simulink model "FsaeDynoFull"  (R2026a)
settings: Solver=FixedStepDiscrete  StopTime=t_stop  FixedStep=Ts  EnableMultiTasking=on
PreLoadFcn:
  | FsaeDynoFullData;
InitFcn:
  | FsaeDynoFullData;
values from neighbouring files (symbols this model uses):
  ce = 100    [FsaeDynoFullData.m]
  k_pre = 0.95    [FsaeDynoFullData.m]    (also in FsaeDynoFullPlot.m = evalin('base','k_pre'))
  Ki_id = Rs*wc_dut    (= 13.3454855924)    [FsaeDynoFullData.m]
  Ki_ids = Rs_y*wc_load    (= 47.1238898038)    [FsaeDynoFullData.m]
  Ki_iq = Rs*wc_dut    (= 13.3454855924)    [FsaeDynoFullData.m]
  Ki_iqs = Rs_y*wc_load    (= 47.1238898038)    [FsaeDynoFullData.m]
  Kp_id = Ld*wc_dut    (= 0.102541584213)    [FsaeDynoFullData.m]
  Kp_ids = Ld_y*wc_load    (= 0.204203522483)    [FsaeDynoFullData.m]
  Kp_iq = Lq*wc_dut    (= 0.105557513161)    [FsaeDynoFullData.m]
  Kp_iqs = Lq_y*wc_load    (= 0.204203522483)    [FsaeDynoFullData.m]
  Ld = 40.8e-6    (= 4.08e-05)    [FsaeDynoFullData.m]
  Lq = 42.0e-6    (= 4.2e-05)    [FsaeDynoFullData.m]
  p = 10    [FsaeDynoFullData.m]    (also in buildFsaeDynoFull.m = get_param(ss,'PortHandles'))
  psim = 0.03095    [FsaeDynoFullData.m]
  R_dis_dut = 1/G_dis_dut  - R_disRly    [FsaeDynoFullData.m]
  R_dis_load = 1/G_dis_load - R_disRly    [FsaeDynoFullData.m]
  R_pre_dut = fzero(@(R) preErr(R, Cdc_dut,  G_leak_dut  + G_disRlyOff), [1 1e5])    [FsaeDynoFullData.m]
  R_pre_load = fzero(@(R) preErr(R, Cdc_load, G_leak_load + G_disRlyOff), [1 1e5])    [FsaeDynoFullData.m]
  R_stby_dut = 50e3    (= 50000)    [FsaeDynoFullData.m]
  R_stby_load = 50e3    (= 50000)    [FsaeDynoFullData.m]
  t_InvEnDelay = 0.05    [FsaeDynoFullData.m]
  t_TSoff = t_test + 0.8 + 0.7    (= 2.7)    [FsaeDynoFullData.m]    (also in FsaeDynoFullPlot.m = evalin('base','t_TSoff'))
  Ts = 1e-5    (= 1e-05)    [FsaeDynoFullData.m]
  VbattMin = 50    [FsaeDynoFullData.m]
  VDC_VECT = Vnom*[0.9 1.0 1.1]    [FsaeDynoFullData.m]
  Vnom2 = 400    [FsaeDynoFullData.m]
libraries: nesl_utility x37, fl_lib x22, ee_lib x22, simulink x4, eeTransforms x2, batteryecm_lib x2, eePmsmFieldOrientedControl x1, eePmsmCurrentController x1, eePmsmCurrentReferenceGen x1, eePmsmTorqueEstimator x1, eePwmGeneratorTwoLevel x1
(part 1 of 2)
CloseFcn:
  | clear simlog_FsaeDyno
  | clear logsout_FsaeDyno
Description:
  | Electric Engine Dyno
settings Model: Creator=The MathWorks, Inc.  LastModifiedBy=micha
settings DataIOCC: MaxDataPoints=90000  SignalLoggingName=logsout_FsaeDynoFull
settings SimscapeCC: SimscapeNominalValues="[{\"value\":\"1\",\"unit\":\"A\"},{\"value\":\"1\",\"unit\":\"bar\"},{\"value\":\"1\",\"unit\":\"cm^2\"},{\"value\":\"1\",\"unit\":\"cm^3/s\"},{\"value\":\"1\",\"unit\":\"kJ/kg\"},{\"value\":\"1\",\"unit\":\"kW\"},{\"value\":\"1\",\"unit\":\"l\"},{\"value\":\"1\",\"unit\":\"N\"},{\"value\":\"1\",\"unit\":\"N*m\"},{\"value\":\"1\",\"unit\":\"V\"}]"  SimscapeLogSimulationStatistics=on  SimscapeLogName=simlog_FsaeDyno  SimscapeLogDataHistory=90000.0

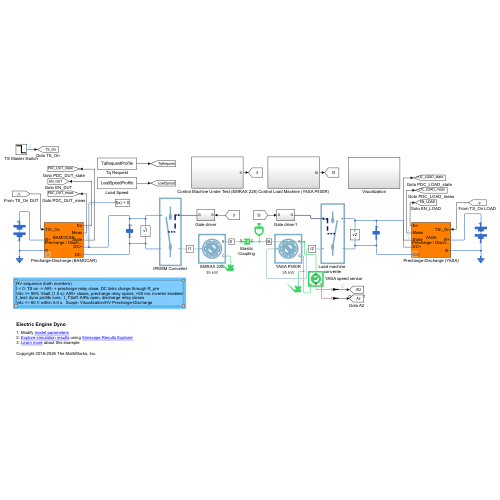
[thumbnail: Simulink's stored preview of the top-level diagram]
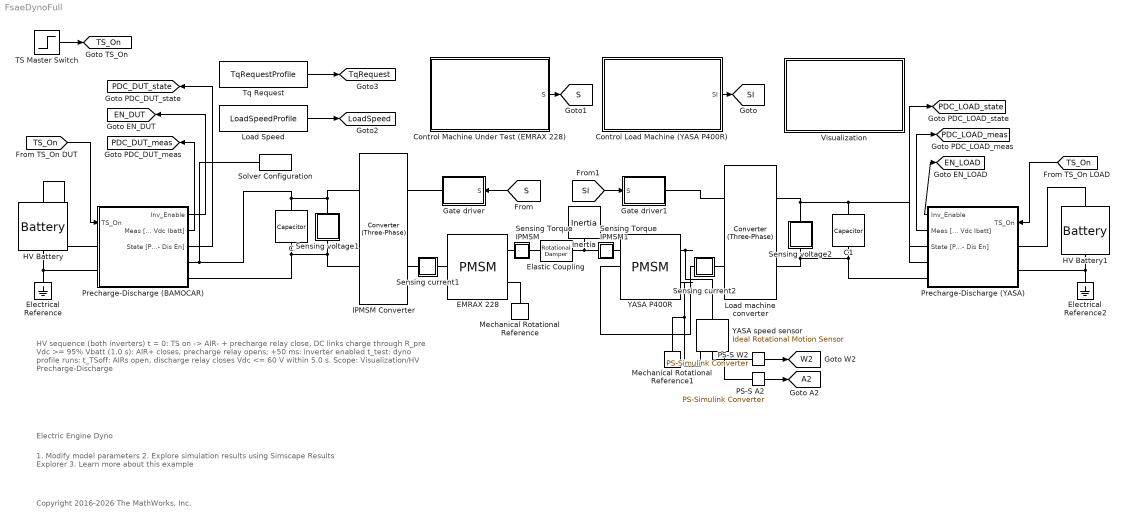
== system FsaeDynoFull ==
  note: Electric Engine Dyno
  note: 1. Modify model parameters
      | 2. Explore simulation results using Simscape Results Explorer
      | 3. Learn more about this example
  note: Copyright 2016-2026 The MathWorks, Inc.
  note: HV sequence (both inverters)
      | t = 0: TS on -> AIR- + precharge relay close, DC links charge through R_pre
      | Vdc >= 95% Vbatt (1.0 s): AIR+ closes, precharge relay opens; +50 ms: inverter enabled
      | t_test: dyno profile runs;  t_TSoff: AIRs open, discharge relay closes
      | Vdc <= 60 V within 5.0 s.  Scope: Visualization/HV Precharge-Discharge
  C : fl_lib/Electrical/Electrical Elements/Capacitor  c=Cdc_dut F  r=1e-6 Ohm  g=0 1/Ohm  i_specify=off  i_priority=None  i=0 A  i_nominal_specify=off  i_nominal_value=1  i_nominal_unit=A  v_specify=off  v_priority=None  v=0 V  v_nominal_specify=off  v_nominal_value=1  v_nominal_unit=V  vc_specify=on  vc_priority=None  vc=0 V  vc_nominal_specify=off  vc_nominal_value=1  vc_nominal_unit=V
  C1 : fl_lib/Electrical/Electrical Elements/Capacitor  c=Cdc_load F  r=1e-6 Ohm  g=0 1/Ohm  i_specify=off  i_priority=None  i=0 A  i_nominal_specify=off  i_nominal_value=1  i_nominal_unit=A  v_specify=off  v_priority=None  v=0 V  v_nominal_specify=off  v_nominal_value=1  v_nominal_unit=V  vc_specify=on  vc_priority=None  vc=0 V  vc_nominal_specify=off  vc_nominal_value=1  vc_nominal_unit=V
  Control Load Machine (YASA P400R) : Subsystem
  Control Machine Under Test (EMRAX 228) : Subsystem
  EMRAX 228 : ee_lib/Electromechanical/Permanent Magnet/PMSM  port_option=ee.enum.threePhasePort.composite  winding_type=ee.enum.statorconnection.wye  machine_param=ee.enum.pmsm.parameterization.constant  nPolePairs=p  pmflux_param=1  pm_flux_linkage=psim Wb  torque_constant=0.18 N*m/A  back_emf_constant=0.18 V/(rad/s)  stator_param=1  Ld=Ld H  Lq=Lq H  idVec=[-200, 0, 200] A  iqVec=[-200, 0, 200] A  LdMatrix=0.0002 * ones(3, 3) H  LqMatrix=0.0002 * ones(3, 3) H  PmMatrix=0.1 * ones(3, 3) Wb  ktMatrix=0.18 * ones(3, 3) N*m/A  keMatrix=0.18 * ones(3, 3) V/(rad/s)  L0=L0 H  Ls=0.0002 H  Lm=0.00002 H  Ms=0.00002 H  Rs=Rs Ohm  zero_sequence=ee.enum.park.zerosequence.exclude  axes_param=ee.enum.rotorangle.qaxis  loss_param=ee.enum.ironloss.none  losses_oc=[0, 0, 0] W  losses_sc=[0, 0, 0] W  f_losses=60 Hz  Isc_losses=95 A  J=0 kg*m^2  lam=0 N*m/(rad/s)  i_d_specify=on  i_d_priority=None  i_d=0 A  i_d_nominal_specify=off  i_d_nominal_value=1  i_d_nominal_unit=A  i_q_specify=on  i_q_priority=None  i_q=0 A  i_q_nominal_specify=off  i_q_nominal_value=1  i_q_nominal_unit=A  torque_specify=off  torque_priority=None  torque=0 N*m  torque_nominal_specify=off  torque_nominal_value=1  torque_nominal_unit=N*m  angular_velocity_specify=off  angular_velocity_priority=None  angular_velocity=0 rpm  angular_velocity_nominal_specify=off  angular_velocity_nominal_value=1  angular_velocity_nominal_unit=rpm  angular_position_specify=on  angular_position_priority=High  angular_position=0 deg  angular_position_nominal_specify=off  angular_position_nominal_value=1  angular_position_nominal_unit=deg  alpha=3.93e-3 1/K  alpha_flux=-0.001 1/K  Tmeas=298.15 K  stator_thermal_mass=100 J/K  rotor_thermal_mass=200 J/K  Rm_percent_rotor=90  Rd_percent_rotor=30  temperatureA_specify=off  temperatureA_priority=High  temperatureA=25 degC  temperatureA_nominal_specify=off  temperatureA_nominal_value=1  temperatureA_nominal_unit=degC  temperatureB_specify=off  temperatureB_priority=High  temperatureB=25 degC  temperatureB_nominal_specify=off  temperatureB_nominal_value=1  temperatureB_nominal_unit=degC  temperatureC_specify=off  temperatureC_priority=High  temperatureC=25 degC  temperatureC_nominal_specify=off  temperatureC_nominal_value=1  temperatureC_nominal_unit=degC  temperatureR_specify=off  temperatureR_priority=High  temperatureR=25 degC  temperatureR_nominal_specify=off  temperatureR_nominal_value=1  temperatureR_nominal_unit=degC
      settings: AttributesFormatString=35 kW
  Elastic Coupling : fl_lib/Mechanical/Rotational Elements/Rotational Damper  D=ce N*m/(rad/s)  w_specify=off  w_priority=None  w=0 rad/s  w_nominal_specify=off  w_nominal_value=1  w_nominal_unit=rad/s  t_specify=off  t_priority=None  t=0 N*m  t_nominal_specify=off  t_nominal_value=1  t_nominal_unit=N*m
      settings: LogSimulationData=on
  Electrical Reference : fl_lib/Electrical/Electrical Elements/Electrical Reference
  Electrical Reference2 : fl_lib/Electrical/Electrical Elements/Electrical Reference
  Gate driver : Subsystem
  Gate driver1 : Subsystem
  HV Battery : batteryecm_lib/Battery  Vnom=Vnom V  prm_dir=1  R1_dis=2 Ohm  R1_ch=2 Ohm  R1=R1_batt Ohm  prm_AH=1  AH=10000 hr*A  V1=V1 V  AH1=3000 hr*A  prm_R2=1  R2=2000 Ohm  Tmeas=298.15 K  charge_measurement_port=simscape.enum.battery.enable.no  prm_dyn=1  Rp1=0.005 Ohm  tau1=30 s  Rp2=0.005 Ohm  tau2=30 s  Rp3=0.005 Ohm  tau3=30 s  Rp4=0.005 Ohm  tau4=30 s  Rp5=0.005 Ohm  tau5=30 s  prm_fade=1  N_fade=100  AH_fade=45 hr*A  R1_fade=2.02 Ohm  R1_ch_fade=2.02 Ohm  V1_fade=10.35 V  prm_age=1  prm_age_OCV=1  OCV_age=0.9  SOC_age=60  Tmeas_age=298.15 K  delta_time_age_vec=[0] d  temperature_age_vec=[273] K  OCV_scaling_age=2.2134e6  OCV_offset_age=1.632e6  temp_exp_age=0.515833569 V  t_exp_age=0.75  Vnom_T2=12 V  R1_T2=2.2 Ohm  R1_T2_dis=2.2 Ohm  R1_T2_ch=2.2 Ohm  V1_T2=11.4 V  R2_T2=2200 Ohm  Rp1_T2=0.005 Ohm  tau1_T2=30 s  Rp2_T2=0.005 Ohm  tau2_T2=30 s  Rp3_T2=0.005 Ohm  tau3_T2=30 s  Rp4_T2=0.005 Ohm  tau4_T2=30 s  Rp5_T2=0.005 Ohm  tau5_T2=30 s  Tmeas2=273.15 K  thermal_port=simscape.enum.thermaleffects.omit  thermal_mass=30000 J/K  i_specify=off  i_priority=None  i=0 A  i_nominal_specify=off  i_nominal_value=1  i_nominal_unit=A  v_specify=off  v_priority=None  v=0 V  v_nominal_specify=off  v_nominal_value=1  v_nominal_unit=V  charge_specify=on  charge_priority=None  charge=8000 hr*A  charge_nominal_specify=off  charge_nominal_value=1  charge_nominal_unit=A*hr  num_cycles_specify=off  num_cycles_priority=High  num_cycles=0  num_cycles_nominal_specify=off  num_cycles_nominal_value=1  num_cycles_nominal_unit=1  temperature_specify=off  temperature_priority=High  temperature=298.15 K  temperature_nominal_specify=off  temperature_nominal_value=1  temperature_nominal_unit=K
  HV Battery1 : batteryecm_lib/Battery  Vnom=Vnom2 V  prm_dir=1  R1_dis=2 Ohm  R1_ch=2 Ohm  R1=R1_batt Ohm  prm_AH=1  AH=25000 hr*A  V1=V1_2 V  AH1=20000 hr*A  prm_R2=1  R2=2000 Ohm  Tmeas=298.15 K  charge_measurement_port=simscape.enum.battery.enable.no  prm_dyn=1  Rp1=0.005 Ohm  tau1=30 s  Rp2=0.005 Ohm  tau2=30 s  Rp3=0.005 Ohm  tau3=30 s  Rp4=0.005 Ohm  tau4=30 s  Rp5=0.005 Ohm  tau5=30 s  prm_fade=1  N_fade=100  AH_fade=45 hr*A  R1_fade=2.02 Ohm  R1_ch_fade=2.02 Ohm  V1_fade=10.35 V  prm_age=1  prm_age_OCV=1  OCV_age=0.9  SOC_age=60  Tmeas_age=298.15 K  delta_time_age_vec=[0] d  temperature_age_vec=[273] K  OCV_scaling_age=2.2134e6  OCV_offset_age=1.632e6  temp_exp_age=0.515833569 V  t_exp_age=0.75  Vnom_T2=12 V  R1_T2=2.2 Ohm  R1_T2_dis=2.2 Ohm  R1_T2_ch=2.2 Ohm  V1_T2=11.4 V  R2_T2=2200 Ohm  Rp1_T2=0.005 Ohm  tau1_T2=30 s  Rp2_T2=0.005 Ohm  tau2_T2=30 s  Rp3_T2=0.005 Ohm  tau3_T2=30 s  Rp4_T2=0.005 Ohm  tau4_T2=30 s  Rp5_T2=0.005 Ohm  tau5_T2=30 s  Tmeas2=273.15 K  thermal_port=simscape.enum.thermaleffects.omit  thermal_mass=30000 J/K  i_specify=off  i_priority=None  i=0 A  i_nominal_specify=off  i_nominal_value=1  i_nominal_unit=A  v_specify=off  v_priority=None  v=0 V  v_nominal_specify=off  v_nominal_value=1  v_nominal_unit=V  charge_specify=on  charge_priority=None  charge=20000 hr*A  charge_nominal_specify=off  charge_nominal_value=1  charge_nominal_unit=A*hr  num_cycles_specify=off  num_cycles_priority=High  num_cycles=0  num_cycles_nominal_specify=off  num_cycles_nominal_value=1  num_cycles_nominal_unit=1  temperature_specify=off  temperature_priority=High  temperature=298.15 K  temperature_nominal_specify=off  temperature_nominal_value=1  temperature_nominal_unit=K
  IPMSM Converter : ee_lib/Semiconductors & Converters/Converters/Converter (Three-Phase)  port_option=ee.enum.threePhasePort.composite  fidelity_option=ee.enum.converters.fidelity.detailed  device_type=3  showThermalPort=false  K=0  Vth=0.5 V  Vgt=1 V  Vgt_off=-1 V  Ih=1 A  Vf=0.8 V  Ron=0.001 Ohm  Rds=0.001 Ohm  Goff=1e-5 1/Ohm  Eon_scalar=22.86e-3 J  Eoff_scalar=17.14e-3 J  Eoff_natural_commutation=10e-3 J  Voff=300 V  Iout_scalar=600 A  onCurrentMeasDelay=0 s  useCurrentFromPreviousCycle=false  useVoltageFromPreviousCycle=false  diode_param=2  diode_Vf=0.8 V  diode_Ron=0.001 Ohm  diode_Goff=1e-5 1/Ohm  diode_C=50 nF  diode_iRM=-235 A  diode_iF=300 A  diode_idot=-50 A/us  diode_trr_param=1  diode_trr_factor=3  diode_trr=15 us  diode_Qrr=1.5e+3 s*uA  diode_rec_loss_model=ee.enum.diode.reverseRecoveryModel.fixed  diode_ErecVal=0 J  diode_scaleWithIandV=false  diode_ErecMat=zeros(2, 3) J  diode_TjrecVec=[298.15, 398.15] K  diode_IfrecVec=[.1, 1, 10] A  diode_IrecVal=10 A  diode_VrecVal=10 V  diode_tFilter=1 / 1000 / 100 s  thermal_network_parameterization=ee.enum.thermalNetworkTopology.external  Rth=[.08, .5] K/W  Rth_Cauer=[.08, .1, .5] K/W  Rth_Foster=[.08, .14, .22, .16] K/W  thermal_mass_parameterization=ee.enum.thermalNetwork.timeconstant  thermal_mass=[.01, .5] J/K  thermal_mass_Cauer=[.01, .1, .5] J/K  thermal_mass_Foster=[.001, .005, .05, .5] J/K  thermal_time_constant=[.001, .2] s  thermal_time_constant_Cauer=[.001, .1, .2] s  thermal_time_constant_Foster=[7e-05, .0007, .01, .08] s  thermal_mass_initial_temperatures=[25, 25] degC  thermal_mass_initial_temperatures_Cauer=[25, 25, 25] degC  junction_thermal_mass=0.01 J/K  Tvec_initial_Foster=[25, 25, 25, 25] degC  snubber_type=0  Cs=1e-7 F  Rs=0.1 Ohm  Vce_loss=[0, 150, 300] V
  Inertia : fl_lib/Mechanical/Rotational Elements/Inertia  inertia=Jm kg*m^2  num_ports=foundation.enum.numPorts2.one  w_specify=off  w_priority=High  w=0 rad/s  w_nominal_specify=off  w_nominal_value=1  w_nominal_unit=rad/s  t_specify=off  t_priority=None  t=0 N*m  t_nominal_specify=off  t_nominal_value=1  t_nominal_unit=N*m
  Load Speed : FromWorkspace  VariableName=LoadSpeedProfile  OutputAfterFinalValue=Holding final value
  Load machine converter : ee_lib/Semiconductors & Converters/Converters/Converter (Three-Phase)  port_option=ee.enum.threePhasePort.composite  fidelity_option=ee.enum.converters.fidelity.detailed  device_type=3  showThermalPort=false  K=0  Vth=0.5 V  Vgt=1 V  Vgt_off=-1 V  Ih=1 A  Vf=0.8 V  Ron=0.001 Ohm  Rds=0.001 Ohm  Goff=1e-5 1/Ohm  Eon_scalar=22.86e-3 J  Eoff_scalar=17.14e-3 J  Eoff_natural_commutation=10e-3 J  Voff=300 V  Iout_scalar=600 A  onCurrentMeasDelay=0 s  useCurrentFromPreviousCycle=false  useVoltageFromPreviousCycle=false  diode_param=2  diode_Vf=0.8 V  diode_Ron=0.001 Ohm  diode_Goff=1e-5 1/Ohm  diode_C=50 nF  diode_iRM=-235 A  diode_iF=300 A  diode_idot=-50 A/us  diode_trr_param=1  diode_trr_factor=3  diode_trr=15 us  diode_Qrr=1.5e+3 s*uA  diode_rec_loss_model=ee.enum.diode.reverseRecoveryModel.fixed  diode_ErecVal=0 J  diode_scaleWithIandV=false  diode_ErecMat=zeros(2, 3) J  diode_TjrecVec=[298.15, 398.15] K  diode_IfrecVec=[.1, 1, 10] A  diode_IrecVal=10 A  diode_VrecVal=10 V  diode_tFilter=1 / 1000 / 100 s  thermal_network_parameterization=ee.enum.thermalNetworkTopology.external  Rth=[.08, .5] K/W  Rth_Cauer=[.08, .1, .5] K/W  Rth_Foster=[.08, .14, .22, .16] K/W  thermal_mass_parameterization=ee.enum.thermalNetwork.timeconstant  thermal_mass=[.01, .5] J/K  thermal_mass_Cauer=[.01, .1, .5] J/K  thermal_mass_Foster=[.001, .005, .05, .5] J/K  thermal_time_constant=[.001, .2] s  thermal_time_constant_Cauer=[.001, .1, .2] s  thermal_time_constant_Foster=[7e-05, .0007, .01, .08] s  thermal_mass_initial_temperatures=[25, 25] degC  thermal_mass_initial_temperatures_Cauer=[25, 25, 25] degC  junction_thermal_mass=0.01 J/K  Tvec_initial_Foster=[25, 25, 25, 25] degC  snubber_type=0  Cs=1e-7 F  Rs=0.1 Ohm  Vce_loss=[0, 150, 300] V
  Mechanical Rotational Reference : fl_lib/Mechanical/Rotational Elements/Mechanical Rotational Reference
  Mechanical Rotational Reference1 : fl_lib/Mechanical/Rotational Elements/Mechanical Rotational Reference
  PS-S A2 : nesl_utility/PS-Simulink Converter  PhysicalDomain=network_engine_domain  SubClassName=ps_output  LeftPortType=input  RightPortType=output  PseudoPeriodic=off  Frequencies=[]  VectorFormat=1-D array  Unit=rad  AffineConversion=off
  PS-S W2 : nesl_utility/PS-Simulink Converter  PhysicalDomain=network_engine_domain  SubClassName=ps_output  LeftPortType=input  RightPortType=output  PseudoPeriodic=off  Frequencies=[]  VectorFormat=1-D array  Unit=rad/s  AffineConversion=off
  Precharge-Discharge (BAMOCAR) : Subsystem  mask(Precharge / Discharge Circuit){Rpre=R_pre_dut, Rdis=R_dis_dut, Rstby=R_stby_dut, kpre=k_pre, tEnable=t_InvEnDelay, VbattMin=VbattMin}
      mask prompts: Rpre "Precharge resistance [Ohm]"; Rdis "Discharge resistance [Ohm]"; Rstby "Standby (bleeder) resistance [Ohm]"; kpre "Precharge-complete threshold [-]"; tEnable "Inverter enable delay after AIR+ [s]"; VbattMin "Minimum valid accumulator voltage [V]"
      mask help:
      | Accumulator isolation (AIR+, AIR-), precharge relay + resistor, inverter-side discharge relay + resistor and bleeder, with the sequencing logic from PrechargeDischargeCircuit_BAMOCAR.
      | TS_On = 1: precharge, close AIR+ at Vdc >= kpre*Vbatt, enable inverter after tEnable.  TS_On = 0: open AIRs, close discharge relay.
      mask Display:
      | disp('BAMOCAR\nPrecharge / Discharge');
      | port_label('LConn',1,'B+'); port_label('LConn',2,'B-');
      | port_label('RConn',1,'DC+'); port_label('RConn',2,'DC-');
      | port_label('input',1,'TS\_On'); port_label('output',1,'En');
      | port_label('output',2,'Meas'); port_label('output',3,'State');
  Precharge-Discharge (YASA) : Subsystem  mask(Precharge / Discharge Circuit){Rpre=R_pre_load, Rdis=R_dis_load, Rstby=R_stby_load, kpre=k_pre, tEnable=t_InvEnDelay, VbattMin=VbattMin}
      mask prompts: Rpre "Precharge resistance [Ohm]"; Rdis "Discharge resistance [Ohm]"; Rstby "Standby (bleeder) resistance [Ohm]"; kpre "Precharge-complete threshold [-]"; tEnable "Inverter enable delay after AIR+ [s]"; VbattMin "Minimum valid accumulator voltage [V]"
      mask help:
      | Accumulator isolation (AIR+, AIR-), precharge relay + resistor, inverter-side discharge relay + resistor and bleeder, with the sequencing logic from PrechargeDischargeCircuit_YASA.
      | TS_On = 1: precharge, close AIR+ at Vdc >= kpre*Vbatt, enable inverter after tEnable.  TS_On = 0: open AIRs, close discharge relay.
      mask Display:
      | disp('YASA\nPrecharge / Discharge');
      | port_label('LConn',1,'B+'); port_label('LConn',2,'B-');
      | port_label('RConn',1,'DC+'); port_label('RConn',2,'DC-');
      | port_label('input',1,'TS\_On'); port_label('output',1,'En');
      | port_label('output',2,'Meas'); port_label('output',3,'State');
  Sensing Torque IPMSM : Subsystem
      mask Display: disp('tI')
  Sensing Torque IPMSM1 : Subsystem
      mask Display: disp('tA')
  Sensing current1 : Subsystem
      mask Display: disp('i1')
  Sensing current2 : Subsystem
      mask Display: disp('i2')
  Sensing voltage1 : Subsystem
      mask Display: disp('v1')
  Sensing voltage2 : Subsystem
      mask Display: disp('v2')
  Solver Configuration : nesl_utility/Solver Configuration  PhysicalDomain=network_engine_domain  SubClassName=solver  LeftPortType=input  RightPortType=generic  Tones=[]  Harmonics=[]  SimulateNoise=off  Profile=off  UseLocalSampling=off  EnableSwitchedLinearOptims=on  FrequencyDomain=off  UseCCode=off  RelTol=0.001  AbsTol=1e-06  MinStep=1e-09  ToWorkspace=off  RevertToSquareIcSolve=off  NumHomotopyIterations=100  PhasorMode=off  PhasorModeNumHarmonics=1  ConsistencySolver=NEWTON_FTOL  CanonicalOrdering=UNORDERED  OptimizeIntermediates=UNOPTIMIZED  IndexReductionMethod=DerivativeReplacement  DoDC=off  ResidualTolerance=1e-9  ConsistencyTolSource=GLOBAL  ConsistencyAbsTol=0.001  ConsistencyRelTol=0.001  ConsistencyTolFactor=0.001  UseLocalSolver=on  LocalSolverChoice=NE_BACKWARD_EULER_ADVANCER  ResolveIndetEquations=on  FunctionEvalNumThread=1  LocalSolverSampleTime=Ts  DoFixedCost=on  MaxNonlinIter=5  MaxModeIter=2  ComputeImpulses=off  ImpulseIterations=2  LinearAlgebra=auto  LinearAlgebraNumThread=0  EquationFormulation=NE_TIME_EF  DelaysMemoryBudget=1024  AutomaticFiltering=on  FilteringTimeConstant=0.001  PartitionStorageMethod=AS_NEEDED  PartitionMemoryBudget=1024  PartitionMethod=FAST  MultibodyUseLocalSolver=off  MultibodyLocalSolverChoice=ODE1  MultibodyLocalSolverSampleTime=0.001
  TS Master Switch : Step  Time=t_TSoff  InitialValue=1  FinalValue=0  SampleTime=Ts
  Tq Request : FromWorkspace  VariableName=TqRequestProfile  OutputAfterFinalValue=Holding final value
  Visualization : Subsystem
  YASA P400R : ee_lib/Electromechanical/Permanent Magnet/PMSM  port_option=ee.enum.threePhasePort.composite  winding_type=ee.enum.statorconnection.wye  machine_param=ee.enum.pmsm.parameterization.constant  nPolePairs=p_y  pmflux_param=1  pm_flux_linkage=psim_y Wb  torque_constant=0.18 N*m/A  back_emf_constant=0.18 V/(rad/s)  stator_param=1  Ld=Ld_y H  Lq=Lq_y H  idVec=[-200, 0, 200] A  iqVec=[-200, 0, 200] A  LdMatrix=0.0002 * ones(3, 3) H  LqMatrix=0.0002 * ones(3, 3) H  PmMatrix=0.1 * ones(3, 3) Wb  ktMatrix=0.18 * ones(3, 3) N*m/A  keMatrix=0.18 * ones(3, 3) V/(rad/s)  L0=Ld_y H  Ls=0.0002 H  Lm=0.00002 H  Ms=0.00002 H  Rs=Rs_y Ohm  zero_sequence=ee.enum.park.zerosequence.exclude  axes_param=ee.enum.rotorangle.qaxis  loss_param=ee.enum.ironloss.none  losses_oc=[0, 0, 0] W  losses_sc=[0, 0, 0] W  f_losses=60 Hz  Isc_losses=95 A  J=0 kg*m^2  lam=0 N*m/(rad/s)  i_d_specify=on  i_d_priority=None  i_d=0 A  i_d_nominal_specify=off  i_d_nominal_value=1  i_d_nominal_unit=A  i_q_specify=on  i_q_priority=None  i_q=0 A  i_q_nominal_specify=off  i_q_nominal_value=1  i_q_nominal_unit=A  torque_specify=off  torque_priority=None  torque=0 N*m  torque_nominal_specify=off  torque_nominal_value=1  torque_nominal_unit=N*m  angular_velocity_specify=off  angular_velocity_priority=None  angular_velocity=0 rpm  angular_velocity_nominal_specify=off  angular_velocity_nominal_value=1  angular_velocity_nominal_unit=rpm  angular_position_specify=on  angular_position_priority=High  angular_position=0 deg  angular_position_nominal_specify=off  angular_position_nominal_value=1  angular_position_nominal_unit=deg  alpha=3.93e-3 1/K  alpha_flux=-0.001 1/K  Tmeas=298.15 K  stator_thermal_mass=100 J/K  rotor_thermal_mass=200 J/K  Rm_percent_rotor=90  Rd_percent_rotor=30  temperatureA_specify=off  temperatureA_priority=High  temperatureA=25 degC  temperatureA_nominal_specify=off  temperatureA_nominal_value=1  temperatureA_nominal_unit=degC  temperatureB_specify=off  temperatureB_priority=High  temperatureB=25 degC  temperatureB_nominal_specify=off  temperatureB_nominal_value=1  temperatureB_nominal_unit=degC  temperatureC_specify=off  temperatureC_priority=High  temperatureC=25 degC  temperatureC_nominal_specify=off  temperatureC_nominal_value=1  temperatureC_nominal_unit=degC  temperatureR_specify=off  temperatureR_priority=High  temperatureR=25 degC  temperatureR_nominal_specify=off  temperatureR_nominal_value=1  temperatureR_nominal_unit=degC
      settings: AttributesFormatString=35 kW
  YASA speed sensor : fl_lib/Mechanical/Mechanical Sensors/Ideal Rotational Motion Sensor  reference=foundation.enum.MeasurementReference.difference  acceleration_port=false  velocity_port=true  position_port=true  wrap_angle=simscape.enum.onoff.off  offset=0 deg
  tag scope: A2=global, EN_DUT=global, EN_LOAD=global, LoadSpeed=global, PDC_DUT_meas=global, PDC_DUT_state=global, PDC_LOAD_meas=global, PDC_LOAD_state=global, S=global, SI=global, TS_On=global, TqRequest=global, W2=global
  wires:
  [S] -> Gate driver/1(S)
  Control Load Machine (YASA P400R)/1(SI) -> [SI]
  Control Machine Under Test (EMRAX 228)/1(S) -> [S]
  [SI] -> Gate driver1/1(S)
  PS-S W2/1 -> [W2]
  PS-S A2/1 -> [A2]
  Load Speed/1 -> [LoadSpeed]
  Tq Request/1 -> [TqRequest]
  TS Master Switch/1 -> [TS_On]
  [TS_On] -> Precharge-Discharge (BAMOCAR)/1(TS_On)
  Precharge-Discharge (BAMOCAR)/1(Inv_Enable) -> [EN_DUT]
  Precharge-Discharge (BAMOCAR)/2(Meas [Vbatt Vdc Ibatt]) -> [PDC_DUT_meas]
  Precharge-Discharge (BAMOCAR)/3(State [Pre AIR+ AIR- Dis En]) -> [PDC_DUT_state]
  [TS_On] -> Precharge-Discharge (YASA)/1(TS_On)
  Precharge-Discharge (YASA)/1(Inv_Enable) -> [EN_LOAD]
  Precharge-Discharge (YASA)/2(Meas [Vbatt Vdc Ibatt]) -> [PDC_LOAD_meas]
  Precharge-Discharge (YASA)/3(State [Pre AIR+ AIR- Dis En]) -> [PDC_LOAD_state]
  connections:
  Gate driver/RConn1 -- IPMSM Converter/LConn1
  EMRAX 228/RConn2 -- Mechanical Rotational Reference/LConn1
  Elastic Coupling/LConn1 -- Sensing Torque IPMSM/RConn1
  IPMSM Converter/LConn2 -- Sensing current1/LConn1
  EMRAX 228/LConn1 -- Sensing current1/RConn1
  Sensing current2/LConn1 -- Load machine converter/LConn2
  Gate driver1/RConn1 -- Load machine converter/LConn1
  Elastic Coupling/RConn1 -- Sensing Torque IPMSM1/LConn1 -- Inertia/LConn1
  Sensing Torque IPMSM/LConn1 -- EMRAX 228/RConn1
  YASA P400R/LConn1 -- Sensing current2/RConn1
  Sensing Torque IPMSM1/RConn1 -- YASA P400R/RConn1 -- YASA speed sensor/LConn1
  Mechanical Rotational Reference1/LConn1 -- YASA P400R/RConn2 -- YASA speed sensor/RConn1
  YASA speed sensor/RConn2 -- PS-S W2/LConn1
  YASA speed sensor/RConn3 -- PS-S A2/LConn1
  HV Battery/LConn1 -- Precharge-Discharge (BAMOCAR)/LConn1
  Precharge-Discharge (BAMOCAR)/LConn2 -- HV Battery/RConn1 -- Electrical Reference/LConn1
  C/LConn1 -- Precharge-Discharge (BAMOCAR)/RConn1 -- Solver Configuration/RConn1 -- Sensing voltage1/LConn1 -- IPMSM Converter/RConn1
  C/RConn1 -- Precharge-Discharge (BAMOCAR)/RConn2 -- Sensing voltage1/RConn1 -- IPMSM Converter/RConn2
  HV Battery1/LConn1 -- Precharge-Discharge (YASA)/LConn1
  Precharge-Discharge (YASA)/LConn2 -- HV Battery1/RConn1 -- Electrical Reference2/LConn1
  C1/LConn1 -- Precharge-Discharge (YASA)/RConn1 -- Sensing voltage2/LConn1 -- Load machine converter/RConn1
  C1/RConn1 -- Precharge-Discharge (YASA)/RConn2 -- Sensing voltage2/RConn1 -- Load machine converter/RConn2

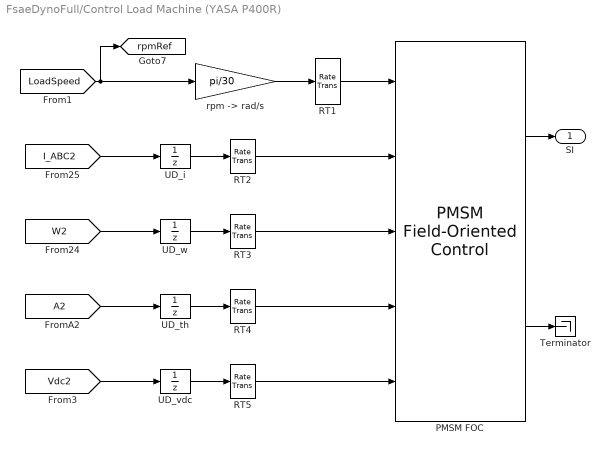
== system FsaeDynoFull/Control Load Machine (YASA P400R) ==
  PMSM FOC : eePmsmFieldOrientedControl/PMSM Field-Oriented Control  winding_type=Wye-wound  CtrlMode=Velocity control  Vnom=Vnom2  Pmax=Pmax_y  Tmax=Tmax_y  p=p_y  Vdc_on=0.5*Vnom2  Ts=Ts  Tsc=Tsc  CtrlType=PI control  Kp_w=Kp_wr  Ki_w=Ki_wr  Kv_w=1  Kaw_w=Kaw_wr  RefType=Zero d-axis control  rpmVec=[0, 3000]  TqVec=[-100, 0, 100]  VdcVec=[300, 350]  PWMMode=SVM: space vector modulation  ModFactor=1  idMatrix=zeros(2,3,2)  iqMatrix=zeros(2,3,2)  psim=psim_y  Ld=Ld_y  Lq=Lq_y  Rs=Rs_y  AxisAlignment=Q-axis  Kp_id=Kp_ids  Ki_id=Ki_ids  Kaw_id=Ki_ids/Kp_ids  Kp_iq=Kp_iqs  Ki_iq=Ki_iqs  Kaw_iq=Ki_iqs/Kp_iqs  AxisPrio=Q-axis  ActZC=off  ActFF=on  ParamTypeFF=Constant parameters  LdFF=Ld_y  LqFF=Lq_y  psimFF=psim_y  idVect=[-200, 0, 200]  iqVect=[-200, 0, 200]  LdMatrix=0.0002 * ones(3, 3)  LqMatrix=0.0002 * ones(3, 3)  psimMatrix=0.04 * ones(3, 3)  CPWMMode=SVM: space vector modulation  fsw=fsw2
  RT{1..5} (5 alike) : RateTransition  OutPortSampleTime=Tsc
  Terminator : Terminator
  UD_i : UnitDelay  SampleTime=Ts
  UD_th : UnitDelay  SampleTime=Ts
  UD_vdc : UnitDelay  SampleTime=Ts
  UD_w : UnitDelay  SampleTime=Ts
  "rpm -> rad/s" : Gain  Gain=pi/30
  SI : Outport  VectorParamsAs1DForOutWhenUnconnected=off
  tag scope: rpmRef=global
  wires:
  [I_ABC2] -> UD_i/1
  [W2] -> UD_w/1
  [A2] -> UD_th/1
  [Vdc2] -> UD_vdc/1
  [LoadSpeed] -> "rpm -> rad/s"/1, [rpmRef]
  PMSM FOC/1 -> SI/1
  PMSM FOC/2 -> Terminator/1
  "rpm -> rad/s"/1 -> RT1/1
  RT1/1 -> PMSM FOC/1
  UD_i/1 -> RT2/1
  RT2/1 -> PMSM FOC/2
  UD_w/1 -> RT3/1
  RT3/1 -> PMSM FOC/3
  UD_th/1 -> RT4/1
  RT4/1 -> PMSM FOC/4
  UD_vdc/1 -> RT5/1
  RT5/1 -> PMSM FOC/5

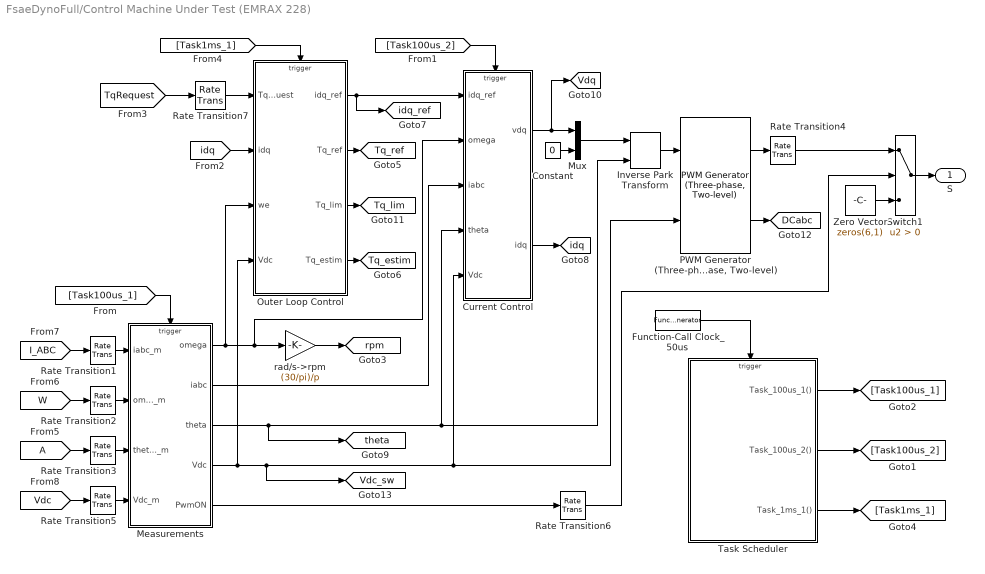
== system FsaeDynoFull/Control Machine Under Test (EMRAX 228) ==
  Constant : Constant  Value=0  SampleTime=-1
  Current Control : Subsystem
  From5 : From  TagVisibility=global
  Function-Call Clock_50us : FunctionCallGenerator  SampleTime=5e-5
  Inverse Park Transform : eeTransforms/Inverse Park Transform  AxisAlignment=Q-axis  PowerInvariant=off
  Measurements : Subsystem
  Mux : Mux  Inputs=2
  Outer Loop Control : Subsystem
  "PWM Generator (Three-phase, Two-level)" : eePwmGeneratorTwoLevel/PWM Generator (Three-phase, Two-level)  PWMMode=Continuous PWM (CPWM)  CPWMMode=SVM: space vector modulation  DPWMMode=60 DPWM: 60 degree discontinuous PWM  fsw=fsw  Ts=Ts
  Rate Transition{1..7} (7 alike) : RateTransition
  Switch1 : Switch  Criteria=u2 > Threshold  SaturateOnIntegerOverflow=off  InputSameDT=off
  Task Scheduler : Stateflow chart  TreatAsAtomicUnit=on
  Zero Vector : Constant  Value=zeros(6,1)  SampleTime=-1
  rad/s->rpm : Gain  Gain=(30/pi)/p
  S : Outport  VectorParamsAs1DForOutWhenUnconnected=off
  tag scope: DCabc=global, Tq_estim=global, Tq_lim=global, Tq_ref=global, Vdc_sw=global, Vdq=global, idq=global, idq_ref=global, rpm=global, theta=global
  wires:
  Current Control/1(vdq) -> [Vdq], Mux/1
  Measurements/2(iabc) -> Current Control/3(iabc)
  Measurements/3(theta) -> [theta], Inverse Park Transform/2, Current Control/4(theta)
  "PWM Generator (Three-phase, Two-level)"/1 -> Rate Transition4/1
  Inverse Park Transform/1 -> "PWM Generator (Three-phase, Two-level)"/1
  [I_ABC] -> Rate Transition1/1
  [W] -> Rate Transition2/1
  From5/1 -> Rate Transition3/1
  [Vdc] -> Rate Transition5/1
  Outer Loop Control/1(idq_ref) -> [idq_ref], Current Control/1(idq_ref)
  "PWM Generator (Three-phase, Two-level)"/2 -> [DCabc]
  Rate Transition1/1 -> Measurements/1(iabc_m)
  Rate Transition2/1 -> Measurements/2(omega_m)
  Rate Transition3/1 -> Measurements/3(theta_m)
  Rate Transition5/1 -> Measurements/4(Vdc_m)
  Function-Call Clock_50us/1 -> Task Scheduler/Trigger
  Task Scheduler/3(Task_1ms_1()) -> [Task1ms_1]
  Task Scheduler/2(Task_100us_2()) -> [Task100us_2]
  Task Scheduler/1(Task_100us_1()) -> [Task100us_1]
  Outer Loop Control/2(Tq_ref) -> [Tq_ref]
  Measurements/1(omega) -> Outer Loop Control/3(we), Current Control/2(omega), rad/s->rpm/1
  rad/s->rpm/1 -> [rpm]
  Outer Loop Control/3(Tq_lim) -> [Tq_lim]
  Rate Transition7/1 -> Outer Loop Control/1(TqRequest)
  [TqRequest] -> Rate Transition7/1
  Outer Loop Control/4(Tq_estim) -> [Tq_estim]
  [idq] -> Outer Loop Control/2(idq)
  Measurements/4(Vdc) -> [Vdc_sw], "PWM Generator (Three-phase, Two-level)"/2, Current Control/5(Vdc), Outer Loop Control/4(Vdc)
  Rate Transition4/1 -> Switch1/1
  Switch1/1 -> S/1
  Measurements/5(PwmON) -> Rate Transition6/1
  Zero Vector/1 -> Switch1/3
  Rate Transition6/1 -> Switch1/2
  [Task100us_2] -> Current Control/Trigger
  [Task1ms_1] -> Outer Loop Control/Trigger
  [Task100us_1] -> Measurements/Trigger
  Current Control/2(idq) -> [idq]
  Constant/1 -> Mux/2
  Mux/1 -> Inverse Park Transform/1

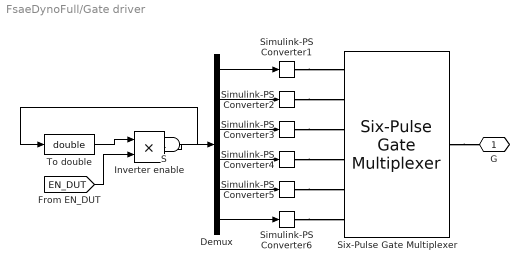
== system FsaeDynoFull/Gate driver ==
  S : Inport
  Demux : Demux  Outputs=6
  Inverter enable : Product  Inputs=**
  Simulink-PS Converter{1..6} (6 alike) : nesl_utility/Simulink-PS Converter  PhysicalDomain=network_engine_domain  SubClassName=ps_input  LeftPortType=input  RightPortType=output  PseudoPeriodic=off  Frequencies=[]  NoiseDistribution=none  NoiseParameters=[]  Unit=1  AffineConversion=off  FilteringAndDerivatives=zero  SimscapeFilterOrder=1  InputFilterTimeConstant=0.001  UdotUserProvided=1
  Six-Pulse Gate Multiplexer : ee_lib/Semiconductors & Converters/Converters/Six-Pulse Gate Multiplexer  port_option=ee.enum.controlport.ps
  To double : DataTypeConversion  OutDataTypeStr=double  SaturateOnIntegerOverflow=off  RndMeth=Floor
  G : PMIOPort  Side=Right
  wires:
  Demux/1 -> Simulink-PS Converter1/1
  Demux/4 -> Simulink-PS Converter4/1
  Demux/2 -> Simulink-PS Converter2/1
  Demux/3 -> Simulink-PS Converter3/1
  Demux/5 -> Simulink-PS Converter5/1
  Demux/6 -> Simulink-PS Converter6/1
  S/1 -> To double/1
  To double/1 -> Inverter enable/1
  [EN_DUT] -> Inverter enable/2
  Inverter enable/1 -> Demux/1
  connections:
  Six-Pulse Gate Multiplexer/RConn1 -- G/RConn1
  Simulink-PS Converter1/RConn1 -- Six-Pulse Gate Multiplexer/LConn1
  Simulink-PS Converter3/RConn1 -- Six-Pulse Gate Multiplexer/LConn3
  Simulink-PS Converter5/RConn1 -- Six-Pulse Gate Multiplexer/LConn5
  Simulink-PS Converter6/RConn1 -- Six-Pulse Gate Multiplexer/LConn6
  Simulink-PS Converter4/RConn1 -- Six-Pulse Gate Multiplexer/LConn4
  Simulink-PS Converter2/RConn1 -- Six-Pulse Gate Multiplexer/LConn2

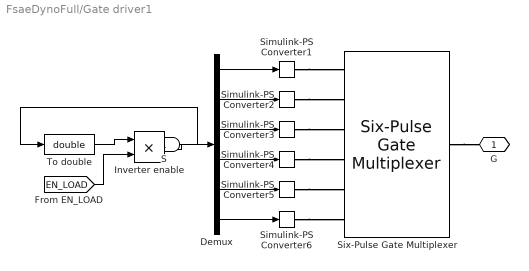
== system FsaeDynoFull/Gate driver1 ==
  S : Inport
  Demux : Demux  Outputs=6
  Inverter enable : Product  Inputs=**
  Simulink-PS Converter{1..6} (6 alike) : nesl_utility/Simulink-PS Converter  PhysicalDomain=network_engine_domain  SubClassName=ps_input  LeftPortType=input  RightPortType=output  PseudoPeriodic=off  Frequencies=[]  NoiseDistribution=none  NoiseParameters=[]  Unit=1  AffineConversion=off  FilteringAndDerivatives=zero  SimscapeFilterOrder=1  InputFilterTimeConstant=0.001  UdotUserProvided=1
  Six-Pulse Gate Multiplexer : ee_lib/Semiconductors & Converters/Converters/Six-Pulse Gate Multiplexer  port_option=ee.enum.controlport.ps
  To double : DataTypeConversion  OutDataTypeStr=double  SaturateOnIntegerOverflow=off  RndMeth=Floor
  G : PMIOPort  Side=Right
  wires:
  Demux/1 -> Simulink-PS Converter1/1
  Demux/4 -> Simulink-PS Converter4/1
  Demux/2 -> Simulink-PS Converter2/1
  Demux/3 -> Simulink-PS Converter3/1
  Demux/5 -> Simulink-PS Converter5/1
  Demux/6 -> Simulink-PS Converter6/1
  S/1 -> To double/1
  To double/1 -> Inverter enable/1
  [EN_LOAD] -> Inverter enable/2
  Inverter enable/1 -> Demux/1
  connections:
  Six-Pulse Gate Multiplexer/RConn1 -- G/RConn1
  Simulink-PS Converter1/RConn1 -- Six-Pulse Gate Multiplexer/LConn1
  Simulink-PS Converter3/RConn1 -- Six-Pulse Gate Multiplexer/LConn3
  Simulink-PS Converter5/RConn1 -- Six-Pulse Gate Multiplexer/LConn5
  Simulink-PS Converter6/RConn1 -- Six-Pulse Gate Multiplexer/LConn6
  Simulink-PS Converter4/RConn1 -- Six-Pulse Gate Multiplexer/LConn4
  Simulink-PS Converter2/RConn1 -- Six-Pulse Gate Multiplexer/LConn2

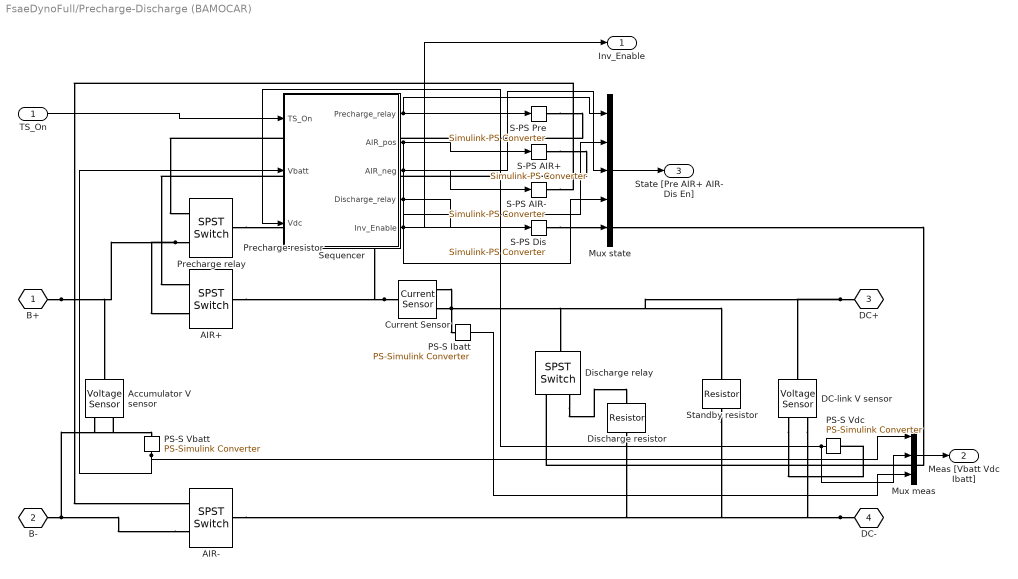
== system FsaeDynoFull/Precharge-Discharge (BAMOCAR) ==
  TS_On : Inport
  AIR+ : ee_lib/Switches & Breakers/SPST Switch  R_closed=0.0003 Ohm  G_open=1e-6 S  Threshold=0.5 V  Width=0 V  model_dynamics=0  t_on=1e-3 s  t_off=1e-3 s  initial_vT=0 V
  AIR- : ee_lib/Switches & Breakers/SPST Switch  R_closed=0.0003 Ohm  G_open=1e-6 S  Threshold=0.5 V  Width=0 V  model_dynamics=0  t_on=1e-3 s  t_off=1e-3 s  initial_vT=0 V
  Accumulator V sensor : fl_lib/Electrical/Electrical Sensors/Voltage Sensor
  Current Sensor : fl_lib/Electrical/Electrical Sensors/Current Sensor
  DC-link V sensor : fl_lib/Electrical/Electrical Sensors/Voltage Sensor
  Discharge relay : ee_lib/Switches & Breakers/SPST Switch  R_closed=0.01 Ohm  G_open=1e-6 S  Threshold=0.5 V  Width=0 V  model_dynamics=0  t_on=1e-3 s  t_off=1e-3 s  initial_vT=0 V
  Discharge resistor : ee_lib/Passive/Resistor  R=Rdis Ohm  enable_R_tol=ee.enum.toleranceApplication.none  R_tol=5  tol_distribution=ee.enum.toleranceDistribution.uniform  nSigma=4  enable_operating_limits=ee.enum.enable.no  operating_limit_action=ee.enum.passive.reportOpLim.warn  power_rating=1 W  max_working_voltage=100 V  noise_mode=ee.enum.sources.noise.Disabled  Tdevice=25 degC  sample_time=1e-3 s  repeatability=ee.enum.ic.repeatability.notRepeatable  user_seed=0  auto_seed=3890346746  power_derating_T1=70 degC  power_derating_T2=155 degC  operating_temperature_range_vec=[-50, 150] degC  alpha=3.93e-3 1/K  Tmeas=25 degC  thermal_mass=100 J/K  temperature_specify=off  temperature_priority=High  temperature=298.15 K  temperature_nominal_specify=off  temperature_nominal_value=1  temperature_nominal_unit=K
  Mux meas : Mux  Inputs=3
  Mux state : Mux  Inputs=5
  PS-S Ibatt : nesl_utility/PS-Simulink Converter  PhysicalDomain=network_engine_domain  SubClassName=ps_output  LeftPortType=input  RightPortType=output  PseudoPeriodic=off  Frequencies=[]  VectorFormat=inherit  Unit=inherit  AffineConversion=off
  PS-S Vbatt : nesl_utility/PS-Simulink Converter  PhysicalDomain=network_engine_domain  SubClassName=ps_output  LeftPortType=input  RightPortType=output  PseudoPeriodic=off  Frequencies=[]  VectorFormat=inherit  Unit=inherit  AffineConversion=off
  PS-S Vdc : nesl_utility/PS-Simulink Converter  PhysicalDomain=network_engine_domain  SubClassName=ps_output  LeftPortType=input  RightPortType=output  PseudoPeriodic=off  Frequencies=[]  VectorFormat=inherit  Unit=inherit  AffineConversion=off
  Precharge relay : ee_lib/Switches & Breakers/SPST Switch  R_closed=0.0003 Ohm  G_open=1e-6 S  Threshold=0.5 V  Width=0 V  model_dynamics=0  t_on=1e-3 s  t_off=1e-3 s  initial_vT=0 V
  Precharge resistor : ee_lib/Passive/Resistor  R=Rpre Ohm  enable_R_tol=ee.enum.toleranceApplication.none  R_tol=5  tol_distribution=ee.enum.toleranceDistribution.uniform  nSigma=4  enable_operating_limits=ee.enum.enable.no  operating_limit_action=ee.enum.passive.reportOpLim.warn  power_rating=1 W  max_working_voltage=100 V  noise_mode=ee.enum.sources.noise.Disabled  Tdevice=25 degC  sample_time=1e-3 s  repeatability=ee.enum.ic.repeatability.notRepeatable  user_seed=0  auto_seed=3499211588  power_derating_T1=70 degC  power_derating_T2=155 degC  operating_temperature_range_vec=[-50, 150] degC  alpha=3.93e-3 1/K  Tmeas=25 degC  thermal_mass=100 J/K  temperature_specify=off  temperature_priority=High  temperature=298.15 K  temperature_nominal_specify=off  temperature_nominal_value=1  temperature_nominal_unit=K
  S-PS AIR+ : nesl_utility/Simulink-PS Converter  PhysicalDomain=network_engine_domain  SubClassName=ps_input  LeftPortType=input  RightPortType=output  PseudoPeriodic=off  Frequencies=[]  NoiseDistribution=none  NoiseParameters=[]  Unit=1  AffineConversion=off  FilteringAndDerivatives=zero  SimscapeFilterOrder=1  InputFilterTimeConstant=0.001  UdotUserProvided=0
  S-PS AIR- : nesl_utility/Simulink-PS Converter  PhysicalDomain=network_engine_domain  SubClassName=ps_input  LeftPortType=input  RightPortType=output  PseudoPeriodic=off  Frequencies=[]  NoiseDistribution=none  NoiseParameters=[]  Unit=1  AffineConversion=off  FilteringAndDerivatives=zero  SimscapeFilterOrder=1  InputFilterTimeConstant=0.001  UdotUserProvided=0
  S-PS Dis : nesl_utility/Simulink-PS Converter  PhysicalDomain=network_engine_domain  SubClassName=ps_input  LeftPortType=input  RightPortType=output  PseudoPeriodic=off  Frequencies=[]  NoiseDistribution=none  NoiseParameters=[]  Unit=1  AffineConversion=off  FilteringAndDerivatives=zero  SimscapeFilterOrder=1  InputFilterTimeConstant=0.001  UdotUserProvided=0
  S-PS Pre : nesl_utility/Simulink-PS Converter  PhysicalDomain=network_engine_domain  SubClassName=ps_input  LeftPortType=input  RightPortType=output  PseudoPeriodic=off  Frequencies=[]  NoiseDistribution=none  NoiseParameters=[]  Unit=1  AffineConversion=off  FilteringAndDerivatives=zero  SimscapeFilterOrder=1  InputFilterTimeConstant=0.001  UdotUserProvided=0
  Sequencer : Subsystem
  Standby resistor : ee_lib/Passive/Resistor  R=Rstby Ohm  enable_R_tol=ee.enum.toleranceApplication.none  R_tol=5  tol_distribution=ee.enum.toleranceDistribution.uniform  nSigma=4  enable_operating_limits=ee.enum.enable.no  operating_limit_action=ee.enum.passive.reportOpLim.warn  power_rating=1 W  max_working_voltage=100 V  noise_mode=ee.enum.sources.noise.Disabled  Tdevice=25 degC  sample_time=1e-3 s  repeatability=ee.enum.ic.repeatability.notRepeatable  user_seed=0  auto_seed=545404223  power_derating_T1=70 degC  power_derating_T2=155 degC  operating_temperature_range_vec=[-50, 150] degC  alpha=3.93e-3 1/K  Tmeas=25 degC  thermal_mass=100 J/K  temperature_specify=off  temperature_priority=High  temperature=298.15 K  temperature_nominal_specify=off  temperature_nominal_value=1  temperature_nominal_unit=K
  B+ : PMIOPort  Side=Left
  B- : PMIOPort  Port=2  Side=Left
  DC+ : PMIOPort  Port=3  Side=Right
  DC- : PMIOPort  Port=4  Side=Right
  Inv_Enable : Outport
  Meas [Vbatt Vdc Ibatt] : Outport  Port=2
  State [Pre AIR+ AIR- Dis En] : Outport  Port=3
  wires:
  TS_On/1 -> Sequencer/1(TS_On)
  PS-S Vbatt/1 -> Sequencer/2(Vbatt), Mux meas/1
  PS-S Vdc/1 -> Sequencer/3(Vdc), Mux meas/2
  Sequencer/1(Precharge_relay) -> S-PS Pre/1, Mux state/1
  Sequencer/2(AIR_pos) -> S-PS AIR+/1, Mux state/2
  Sequencer/3(AIR_neg) -> S-PS AIR-/1, Mux state/3
  Sequencer/4(Discharge_relay) -> S-PS Dis/1, Mux state/4
  Sequencer/5(Inv_Enable) -> Inv_Enable/1, Mux state/5
  Mux state/1 -> State [Pre AIR+ AIR- Dis En]/1
  PS-S Ibatt/1 -> Mux meas/3
  Mux meas/1 -> Meas [Vbatt Vdc Ibatt]/1
  connections:
  Precharge relay/LConn2 -- B+/RConn1 -- Accumulator V sensor/LConn1 -- AIR+/LConn2
  Precharge relay/RConn1 -- Precharge resistor/LConn1
  AIR-/LConn2 -- B-/RConn1 -- Accumulator V sensor/RConn2
  Current Sensor/LConn1 -- Precharge resistor/RConn1 -- AIR+/RConn1
  Current Sensor/RConn2 -- Discharge relay/RConn1 -- Standby resistor/LConn1 -- DC+/RConn1 -- DC-link V sensor/LConn1
  AIR-/RConn1 -- Discharge resistor/RConn1 -- Standby resistor/RConn1 -- DC-/RConn1 -- DC-link V sensor/RConn2
  Discharge relay/LConn2 -- Discharge resistor/LConn1
  Accumulator V sensor/RConn1 -- PS-S Vbatt/LConn1
  DC-link V sensor/RConn1 -- PS-S Vdc/LConn1
  Current Sensor/RConn1 -- PS-S Ibatt/LConn1
  S-PS Pre/RConn1 -- Precharge relay/LConn1
  S-PS AIR+/RConn1 -- AIR+/LConn1
  S-PS AIR-/RConn1 -- AIR-/LConn1
  S-PS Dis/RConn1 -- Discharge relay/LConn1

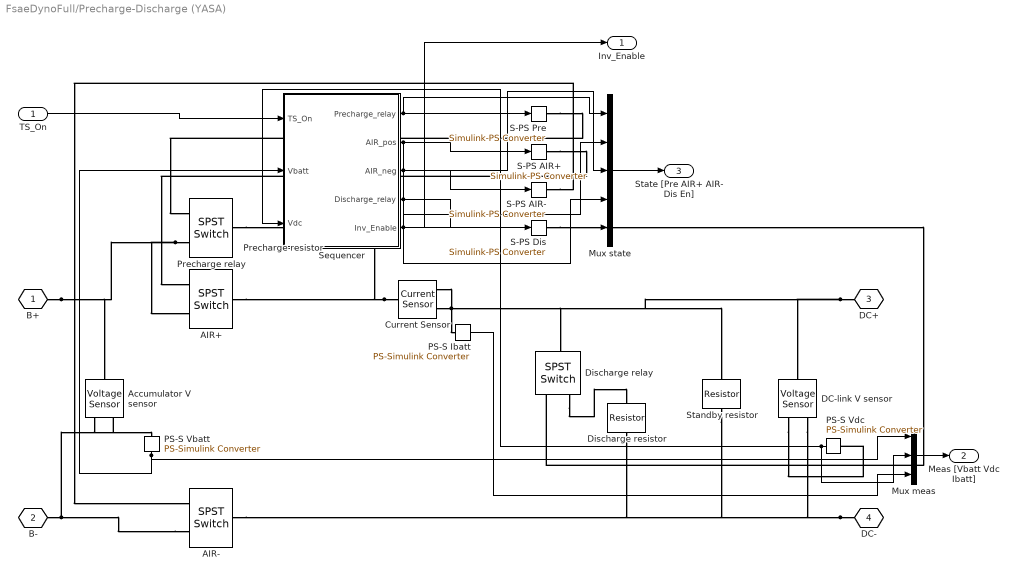
== system FsaeDynoFull/Precharge-Discharge (YASA) ==
  TS_On : Inport
  AIR+ : ee_lib/Switches & Breakers/SPST Switch  R_closed=0.0003 Ohm  G_open=1e-6 S  Threshold=0.5 V  Width=0 V  model_dynamics=0  t_on=1e-3 s  t_off=1e-3 s  initial_vT=0 V
  AIR- : ee_lib/Switches & Breakers/SPST Switch  R_closed=0.0003 Ohm  G_open=1e-6 S  Threshold=0.5 V  Width=0 V  model_dynamics=0  t_on=1e-3 s  t_off=1e-3 s  initial_vT=0 V
  Accumulator V sensor : fl_lib/Electrical/Electrical Sensors/Voltage Sensor
  Current Sensor : fl_lib/Electrical/Electrical Sensors/Current Sensor
  DC-link V sensor : fl_lib/Electrical/Electrical Sensors/Voltage Sensor
  Discharge relay : ee_lib/Switches & Breakers/SPST Switch  R_closed=0.01 Ohm  G_open=1e-6 S  Threshold=0.5 V  Width=0 V  model_dynamics=0  t_on=1e-3 s  t_off=1e-3 s  initial_vT=0 V
  Discharge resistor : ee_lib/Passive/Resistor  R=Rdis Ohm  enable_R_tol=ee.enum.toleranceApplication.none  R_tol=5  tol_distribution=ee.enum.toleranceDistribution.uniform  nSigma=4  enable_operating_limits=ee.enum.enable.no  operating_limit_action=ee.enum.passive.reportOpLim.warn  power_rating=1 W  max_working_voltage=100 V  noise_mode=ee.enum.sources.noise.Disabled  Tdevice=25 degC  sample_time=1e-3 s  repeatability=ee.enum.ic.repeatability.notRepeatable  user_seed=0  auto_seed=2715962282  power_derating_T1=70 degC  power_derating_T2=155 degC  operating_temperature_range_vec=[-50, 150] degC  alpha=3.93e-3 1/K  Tmeas=25 degC  thermal_mass=100 J/K  temperature_specify=off  temperature_priority=High  temperature=298.15 K  temperature_nominal_specify=off  temperature_nominal_value=1  temperature_nominal_unit=K
  Mux meas : Mux  Inputs=3
  Mux state : Mux  Inputs=5
  PS-S Ibatt : nesl_utility/PS-Simulink Converter  PhysicalDomain=network_engine_domain  SubClassName=ps_output  LeftPortType=input  RightPortType=output  PseudoPeriodic=off  Frequencies=[]  VectorFormat=inherit  Unit=inherit  AffineConversion=off
  PS-S Vbatt : nesl_utility/PS-Simulink Converter  PhysicalDomain=network_engine_domain  SubClassName=ps_output  LeftPortType=input  RightPortType=output  PseudoPeriodic=off  Frequencies=[]  VectorFormat=inherit  Unit=inherit  AffineConversion=off
  PS-S Vdc : nesl_utility/PS-Simulink Converter  PhysicalDomain=network_engine_domain  SubClassName=ps_output  LeftPortType=input  RightPortType=output  PseudoPeriodic=off  Frequencies=[]  VectorFormat=inherit  Unit=inherit  AffineConversion=off
  Precharge relay : ee_lib/Switches & Breakers/SPST Switch  R_closed=0.0003 Ohm  G_open=1e-6 S  Threshold=0.5 V  Width=0 V  model_dynamics=0  t_on=1e-3 s  t_off=1e-3 s  initial_vT=0 V
  Precharge resistor : ee_lib/Passive/Resistor  R=Rpre Ohm  enable_R_tol=ee.enum.toleranceApplication.none  R_tol=5  tol_distribution=ee.enum.toleranceDistribution.uniform  nSigma=4  enable_operating_limits=ee.enum.enable.no  operating_limit_action=ee.enum.passive.reportOpLim.warn  power_rating=1 W  max_working_voltage=100 V  noise_mode=ee.enum.sources.noise.Disabled  Tdevice=25 degC  sample_time=1e-3 s  repeatability=ee.enum.ic.repeatability.notRepeatable  user_seed=0  auto_seed=3922919431  power_derating_T1=70 degC  power_derating_T2=155 degC  operating_temperature_range_vec=[-50, 150] degC  alpha=3.93e-3 1/K  Tmeas=25 degC  thermal_mass=100 J/K  temperature_specify=off  temperature_priority=High  temperature=298.15 K  temperature_nominal_specify=off  temperature_nominal_value=1  temperature_nominal_unit=K
  S-PS AIR+ : nesl_utility/Simulink-PS Converter  PhysicalDomain=network_engine_domain  SubClassName=ps_input  LeftPortType=input  RightPortType=output  PseudoPeriodic=off  Frequencies=[]  NoiseDistribution=none  NoiseParameters=[]  Unit=1  AffineConversion=off  FilteringAndDerivatives=zero  SimscapeFilterOrder=1  InputFilterTimeConstant=0.001  UdotUserProvided=0
  S-PS AIR- : nesl_utility/Simulink-PS Converter  PhysicalDomain=network_engine_domain  SubClassName=ps_input  LeftPortType=input  RightPortType=output  PseudoPeriodic=off  Frequencies=[]  NoiseDistribution=none  NoiseParameters=[]  Unit=1  AffineConversion=off  FilteringAndDerivatives=zero  SimscapeFilterOrder=1  InputFilterTimeConstant=0.001  UdotUserProvided=0
  S-PS Dis : nesl_utility/Simulink-PS Converter  PhysicalDomain=network_engine_domain  SubClassName=ps_input  LeftPortType=input  RightPortType=output  PseudoPeriodic=off  Frequencies=[]  NoiseDistribution=none  NoiseParameters=[]  Unit=1  AffineConversion=off  FilteringAndDerivatives=zero  SimscapeFilterOrder=1  InputFilterTimeConstant=0.001  UdotUserProvided=0
  S-PS Pre : nesl_utility/Simulink-PS Converter  PhysicalDomain=network_engine_domain  SubClassName=ps_input  LeftPortType=input  RightPortType=output  PseudoPeriodic=off  Frequencies=[]  NoiseDistribution=none  NoiseParameters=[]  Unit=1  AffineConversion=off  FilteringAndDerivatives=zero  SimscapeFilterOrder=1  InputFilterTimeConstant=0.001  UdotUserProvided=0
  Sequencer : Subsystem
  Standby resistor : ee_lib/Passive/Resistor  R=Rstby Ohm  enable_R_tol=ee.enum.toleranceApplication.none  R_tol=5  tol_distribution=ee.enum.toleranceDistribution.uniform  nSigma=4  enable_operating_limits=ee.enum.enable.no  operating_limit_action=ee.enum.passive.reportOpLim.warn  power_rating=1 W  max_working_voltage=100 V  noise_mode=ee.enum.sources.noise.Disabled  Tdevice=25 degC  sample_time=1e-3 s  repeatability=ee.enum.ic.repeatability.notRepeatable  user_seed=0  auto_seed=418932850  power_derating_T1=70 degC  power_derating_T2=155 degC  operating_temperature_range_vec=[-50, 150] degC  alpha=3.93e-3 1/K  Tmeas=25 degC  thermal_mass=100 J/K  temperature_specify=off  temperature_priority=High  temperature=298.15 K  temperature_nominal_specify=off  temperature_nominal_value=1  temperature_nominal_unit=K
  B+ : PMIOPort  Side=Left
  B- : PMIOPort  Port=2  Side=Left
  DC+ : PMIOPort  Port=3  Side=Right
  DC- : PMIOPort  Port=4  Side=Right
  Inv_Enable : Outport
  Meas [Vbatt Vdc Ibatt] : Outport  Port=2
  State [Pre AIR+ AIR- Dis En] : Outport  Port=3
  wires:
  TS_On/1 -> Sequencer/1(TS_On)
  PS-S Vbatt/1 -> Sequencer/2(Vbatt), Mux meas/1
  PS-S Vdc/1 -> Sequencer/3(Vdc), Mux meas/2
  Sequencer/1(Precharge_relay) -> S-PS Pre/1, Mux state/1
  Sequencer/2(AIR_pos) -> S-PS AIR+/1, Mux state/2
  Sequencer/3(AIR_neg) -> S-PS AIR-/1, Mux state/3
  Sequencer/4(Discharge_relay) -> S-PS Dis/1, Mux state/4
  Sequencer/5(Inv_Enable) -> Inv_Enable/1, Mux state/5
  Mux state/1 -> State [Pre AIR+ AIR- Dis En]/1
  PS-S Ibatt/1 -> Mux meas/3
  Mux meas/1 -> Meas [Vbatt Vdc Ibatt]/1
  connections:
  Precharge relay/LConn2 -- B+/RConn1 -- Accumulator V sensor/LConn1 -- AIR+/LConn2
  Precharge relay/RConn1 -- Precharge resistor/LConn1
  AIR-/LConn2 -- B-/RConn1 -- Accumulator V sensor/RConn2
  Current Sensor/LConn1 -- Precharge resistor/RConn1 -- AIR+/RConn1
  Current Sensor/RConn2 -- Discharge relay/RConn1 -- Standby resistor/LConn1 -- DC+/RConn1 -- DC-link V sensor/LConn1
  AIR-/RConn1 -- Discharge resistor/RConn1 -- Standby resistor/RConn1 -- DC-/RConn1 -- DC-link V sensor/RConn2
  Discharge relay/LConn2 -- Discharge resistor/LConn1
  Accumulator V sensor/RConn1 -- PS-S Vbatt/LConn1
  DC-link V sensor/RConn1 -- PS-S Vdc/LConn1
  Current Sensor/RConn1 -- PS-S Ibatt/LConn1
  S-PS Pre/RConn1 -- Precharge relay/LConn1
  S-PS AIR+/RConn1 -- AIR+/LConn1
  S-PS AIR-/RConn1 -- AIR-/LConn1
  S-PS Dis/RConn1 -- Discharge relay/LConn1
